simulink model "day1"  (R2024a)
settings: Solver=VariableStepAuto  StartTime=0.0  StopTime=4  RelTol=1e-3
settings Model: Creator=user  LastModifiedBy=user

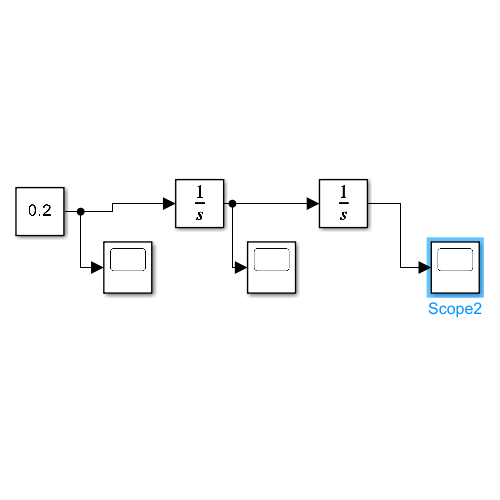
[thumbnail: Simulink's stored preview of the top-level diagram]
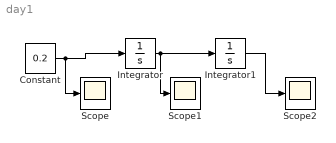
== system day1 ==
  Constant : Constant  Value=0.2  SampleTime=0.002
  Integrator : Integrator  ContinuousStateAttributes="\"velocity\""
  Integrator1 : Integrator  ContinuousStateAttributes="\"altitude\""
  Scope : Scope
  Scope1 : Scope
  Scope2 : Scope
  wires:
  Constant/1 -> Scope/1, Integrator/1
  Integrator/1 -> Scope1/1, Integrator1/1
  Integrator1/1 -> Scope2/1
